simulink model "linearAirframe"  (R2026a)
settings: Solver=ode3  FixedStep=Ts  EnableMultiTasking=on
InitFcn:
  | load('linearizedAirframe.mat');
values from neighbouring files (symbols this model uses):
  linsys = linearize(modelTrim,io,op, linopt)    [trimLinearizeOpPoint.m]
undefined symbols (not defined in the file or in its folder): opreport
settings Model: Creator=The MathWorks, Inc.  LastModifiedBy=The MathWorks, Inc.
settings HardwareCC: ProdHWDeviceType=32-bit Generic

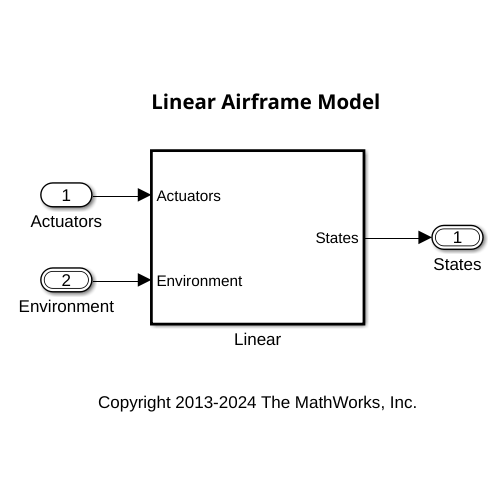
[thumbnail: Simulink's stored preview of the top-level diagram]
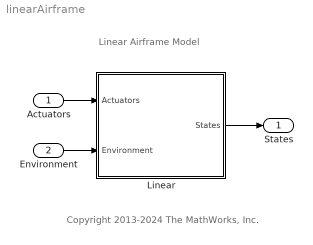
== system linearAirframe ==
  note: Copyright 2013-2024 The MathWorks, Inc.
  note: Linear Airframe Model
  Actuators : Inport  OutDataTypeStr=single  PortDimensions=4
  Environment : Inport  Port=2  OutDataTypeStr=Bus: EnvironmentBus  BusOutputAsStruct=on
  Linear : Subsystem  TreatAsAtomicUnit=on
  States : Outport  OutDataTypeStr=Bus: StatesBus  VectorParamsAs1DForOutWhenUnconnected=off  BusOutputAsStruct=on
  wires:
  Actuators/1 -> Linear/1(Actuators)
  Environment/1 -> Linear/2(Environment)
  Linear/1(States) -> States/1

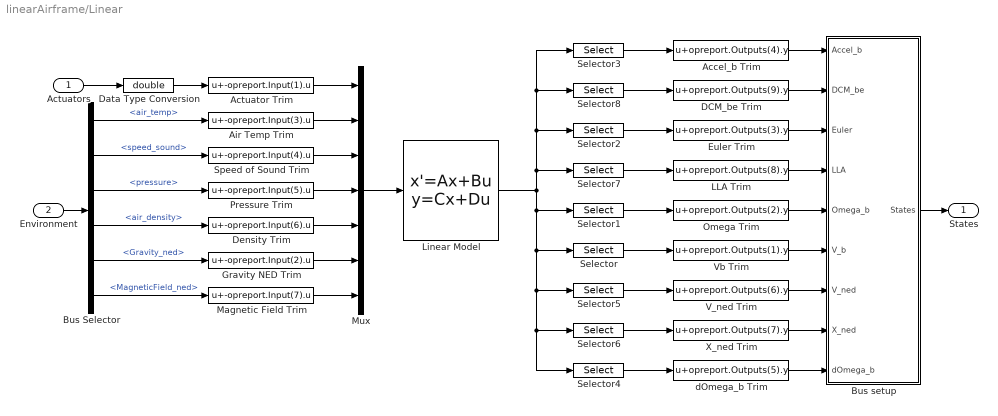
== system linearAirframe/Linear ==
  Actuators : Inport
  Environment : Inport  Port=2  OutDataTypeStr=Bus: EnvironmentBus
  Accel_b Trim : Bias  Bias=opreport.Outputs(4).y  SaturateOnIntegerOverflow=off
  Actuator Trim : Bias  Bias=-opreport.Input(1).u  SaturateOnIntegerOverflow=off
  Air Temp Trim : Bias  Bias=-opreport.Input(3).u  SaturateOnIntegerOverflow=off
  Bus Selector : BusSelector  OutputSignals=AtmosphereBus.air_temp,AtmosphereBus.speed_sound,AtmosphereBus.pressure,AtmosphereBus.air_density,Gravity_ned,MagneticField_ned
  Bus setup : Subsystem
  DCM_be Trim : Bias  Bias=opreport.Outputs(9).y  SaturateOnIntegerOverflow=off
  Data Type Conversion : DataTypeConversion  OutDataTypeStr=double  SaturateOnIntegerOverflow=off  RndMeth=Floor
  Density Trim : Bias  Bias=-opreport.Input(6).u  SaturateOnIntegerOverflow=off
  Euler Trim : Bias  Bias=opreport.Outputs(3).y  SaturateOnIntegerOverflow=off
  Gravity NED Trim : Bias  Bias=-opreport.Input(2).u  SaturateOnIntegerOverflow=off
  LLA Trim : Bias  Bias=opreport.Outputs(8).y  SaturateOnIntegerOverflow=off
  Linear Model : StateSpace  A=linsys.a  B=linsys.b  C=linsys.c  D=linsys.d  InitialCondition=zeros(length(linsys.a),1)
  Magnetic Field Trim : Bias  Bias=-opreport.Input(7).u  SaturateOnIntegerOverflow=off
  Mux : Mux  Inputs=7
  Omega Trim : Bias  Bias=opreport.Outputs(2).y  SaturateOnIntegerOverflow=off
  Pressure Trim : Bias  Bias=-opreport.Input(5).u  SaturateOnIntegerOverflow=off
  Selector : Selector  InputPortWidth=33  IndexOptions=Index vector (dialog)  Indices=[22 23 24]  OutputSizes=1
  Selector1 : Selector  InputPortWidth=33  IndexOptions=Index vector (dialog)  Indices=[19 20 21]  OutputSizes=1
  Selector2 : Selector  InputPortWidth=33  IndexOptions=Index vector (dialog)  Indices=[13 14 15]  OutputSizes=1
  Selector3 : Selector  InputPortWidth=33  IndexOptions=Index vector (dialog)  Indices=[1 2 3]  OutputSizes=1
  Selector4 : Selector  InputPortWidth=33  IndexOptions=Index vector (dialog)  Indices=[31 32 33]  OutputSizes=1
  Selector5 : Selector  InputPortWidth=33  IndexOptions=Index vector (dialog)  Indices=[25 26 27]  OutputSizes=1
  Selector6 : Selector  InputPortWidth=33  IndexOptions=Index vector (dialog)  Indices=[28 29 30]  OutputSizes=1
  Selector7 : Selector  InputPortWidth=33  IndexOptions=Index vector (dialog)  Indices=[16 17 18]  OutputSizes=1
  Selector8 : Selector  InputPortWidth=33  IndexOptions=Index vector (dialog)  Indices=[4 5 6 7 8 9 10 11 12]  OutputSizes=1
  Speed of Sound Trim : Bias  Bias=-opreport.Input(4).u  SaturateOnIntegerOverflow=off
  V_ned Trim : Bias  Bias=opreport.Outputs(6).y  SaturateOnIntegerOverflow=off
  Vb Trim : Bias  Bias=opreport.Outputs(1).y  SaturateOnIntegerOverflow=off
  X_ned Trim : Bias  Bias=opreport.Outputs(7).y  SaturateOnIntegerOverflow=off
  dOmega_b Trim : Bias  Bias=opreport.Outputs(5).y  SaturateOnIntegerOverflow=off
  States : Outport  OutDataTypeStr=Bus: StatesBus  VectorParamsAs1DForOutWhenUnconnected=off
  wires:
  Mux/1 -> Linear Model/1
  Linear Model/1 -> Selector3/1, Selector8/1, Selector2/1, Selector7/1, Selector4/1, Selector6/1, Selector5/1, Selector/1, Selector1/1
  Actuators/1 -> Data Type Conversion/1
  Environment/1 -> Bus Selector/1
  Actuator Trim/1 -> Mux/1
  Bus Selector/5 -> Gravity NED Trim/1  "<Gravity_ned>"
  Bus Selector/1 -> Air Temp Trim/1  "<air_temp>"
  Bus Selector/2 -> Speed of Sound Trim/1  "<speed_sound>"
  Bus Selector/3 -> Pressure Trim/1  "<pressure>"
  Bus Selector/4 -> Density Trim/1  "<air_density>"
  Bus Selector/6 -> Magnetic Field Trim/1  "<MagneticField_ned>"
  Bus setup/1(States) -> States/1
  Selector/1 -> Vb Trim/1
  Selector1/1 -> Omega Trim/1
  Selector2/1 -> Euler Trim/1
  Selector3/1 -> Accel_b Trim/1
  Selector4/1 -> dOmega_b Trim/1
  Selector5/1 -> V_ned Trim/1
  Selector6/1 -> X_ned Trim/1
  Selector7/1 -> LLA Trim/1
  Selector8/1 -> DCM_be Trim/1
  Data Type Conversion/1 -> Actuator Trim/1
  Air Temp Trim/1 -> Mux/2
  Speed of Sound Trim/1 -> Mux/3
  Pressure Trim/1 -> Mux/4
  Density Trim/1 -> Mux/5
  Gravity NED Trim/1 -> Mux/6
  Magnetic Field Trim/1 -> Mux/7
  LLA Trim/1 -> Bus setup/4(LLA)
  dOmega_b Trim/1 -> Bus setup/9(dOmega_b)
  X_ned Trim/1 -> Bus setup/8(X_ned)
  V_ned Trim/1 -> Bus setup/7(V_ned)
  Vb Trim/1 -> Bus setup/6(V_b)
  Omega Trim/1 -> Bus setup/5(Omega_b)
  Euler Trim/1 -> Bus setup/3(Euler)
  DCM_be Trim/1 -> Bus setup/2(DCM_be)
  Accel_b Trim/1 -> Bus setup/1(Accel_b)

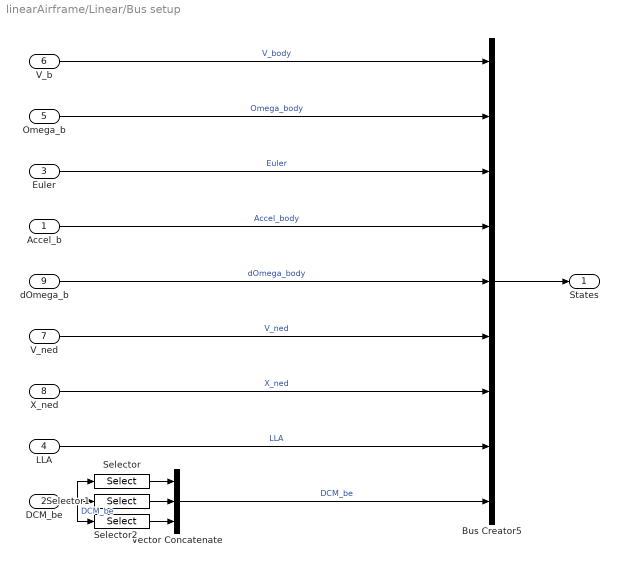
== system linearAirframe/Linear/Bus setup ==
  Accel_b : Inport  Unit=m/s^2  PortDimensions=3
  DCM_be : Inport  Port=2  PortDimensions=9
  Euler : Inport  Port=3  Unit=rad  PortDimensions=3
  LLA : Inport  Port=4  PortDimensions=3
  Omega_b : Inport  Port=5  Unit=rad/s  PortDimensions=3
  V_b : Inport  Port=6  Unit=m/s  PortDimensions=3
  V_ned : Inport  Port=7  Unit=m/second  PortDimensions=3
  X_ned : Inport  Port=8  Unit=m  PortDimensions=3
  dOmega_b : Inport  Port=9  Unit=rad/s^2  PortDimensions=3
  Bus Creator5 : BusCreator  Inputs=9  OutDataTypeStr=Bus: StatesBus  NonVirtualBus=on
  Selector : Selector  InputPortWidth=9  IndexOptions=Index vector (dialog)  Indices=[1 2 3]  OutputSizes=1
  Selector1 : Selector  InputPortWidth=9  IndexOptions=Index vector (dialog)  Indices=[4 5 6]  OutputSizes=1
  Selector2 : Selector  InputPortWidth=9  IndexOptions=Index vector (dialog)  Indices=[7 8 9]  OutputSizes=1
  Vector Concatenate : Concatenate  NumInputs=3  Mode=Multidimensional array  ConcatenateDimension=2
  States : Outport  VectorParamsAs1DForOutWhenUnconnected=off
  wires:
  Bus Creator5/1 -> States/1
  V_b/1 -> Bus Creator5/1  "V_body"
  Omega_b/1 -> Bus Creator5/2  "Omega_body"
  Euler/1 -> Bus Creator5/3  "Euler"
  X_ned/1 -> Bus Creator5/7  "X_ned"
  Accel_b/1 -> Bus Creator5/4  "Accel_body"
  LLA/1 -> Bus Creator5/8  "LLA"
  dOmega_b/1 -> Bus Creator5/5  "dOmega_body"
  Vector Concatenate/1 -> Bus Creator5/9  "DCM_be"
  V_ned/1 -> Bus Creator5/6  "V_ned"
  Selector1/1 -> Vector Concatenate/2
  Selector2/1 -> Vector Concatenate/3
  Selector/1 -> Vector Concatenate/1
  DCM_be/1 -> Selector2/1, Selector1/1, Selector/1  "DCM_be"
